simulink model "r2_b8a4x1kf"  (R2012b)
settings: Solver=VariableStepDiscrete  SolverMode=SingleTasking  StartTime=0.0  StopTime=1  RelTol=1e-3
undefined symbols (not defined in the file): fft_stages, n_bits_ants, n_bits_xengs
libraries: xbsIndex_r4 x22142, casper_library_misc x166, xbsReplacements_r4 x24, casper_library_delays x8, xps_library x5, casper_library_communications x4
(part 20 of 178)

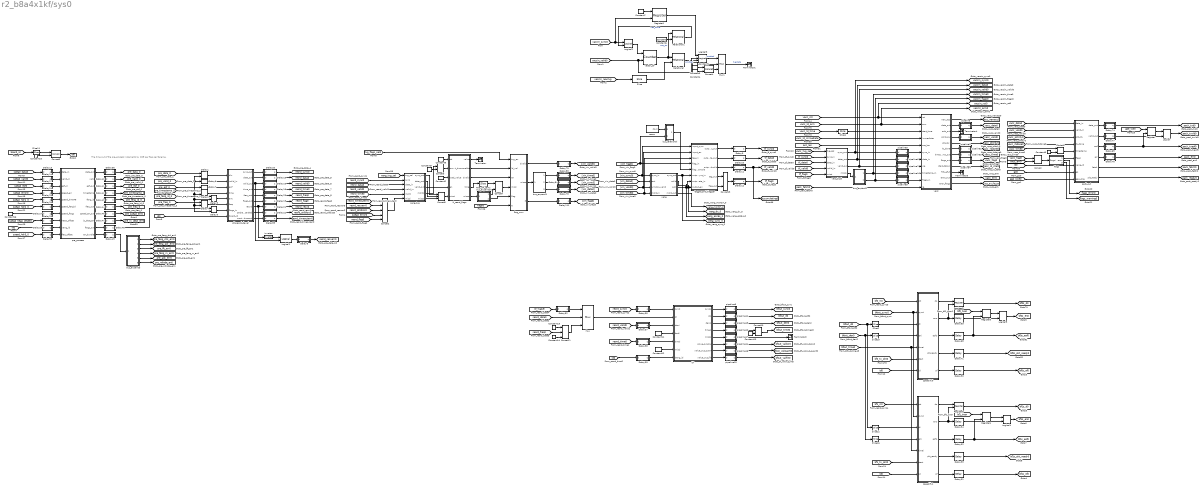
== system r2_b8a4x1kf/sys0 ==
  note: The time out of the pre_process increments
      | by ONE per freq per fengine.
  Concat{,1,3..4,6..7,10,13} (8 alike) : xbsIndex_r4/Concat  num_inputs=2  dbl_ovrd=off  block_type=concat
      Concat1 settings: block_version=10.1.3
      Concat4 settings: block_version=10.1.3
  Concat11 : xbsIndex_r4/Concat  num_inputs=3  dbl_ovrd=off  block_type=concat
  Concat2 : xbsIndex_r4/Concat  num_inputs=5  dbl_ovrd=off  block_type=concat
  Concat5 : xbsIndex_r4/Concat  num_inputs=3  dbl_ovrd=off  block_type=concat
  Constant1 : xbsIndex_r4/Constant  const=0  gui_display_data_type=Fixed-point  arith_type=Unsigned  n_bits=64  bin_pt=0  preci_type=Single  exp_width=8  frac_width=24  explicit_period=on  period=1  equ=P=C  opselect=C  inp2=PCIN>>17  opr=+  inp1=P  carry=CIN  dbl_ovrd=off  block_type=constant
  Constant10 : xbsIndex_r4/Constant  const=xeng_id  gui_display_data_type=Fixed-point  arith_type=Unsigned  n_bits=n_bits_xengs_per_fpga  bin_pt=0  preci_type=Single  exp_width=8  frac_width=24  explicit_period=on  period=1  equ=P=C  opselect=C  inp2=PCIN>>17  opr=+  inp1=P  carry=CIN  dbl_ovrd=off  block_type=constant
  Constant11 : xbsIndex_r4/Constant  const=0  gui_display_data_type=Fixed-point  arith_type=Boolean  n_bits=1  bin_pt=0  preci_type=Single  exp_width=8  frac_width=24  explicit_period=on  period=1  equ=P=C  opselect=C  inp2=PCIN>>17  opr=+  inp1=P  carry=CIN  dbl_ovrd=off  block_type=constant
      settings: block_version=11.3
  Constant12 : xbsIndex_r4/Constant  const=0  gui_display_data_type=Fixed-point  arith_type=Boolean  n_bits=1  bin_pt=0  preci_type=Single  exp_width=8  frac_width=24  explicit_period=on  period=1  equ=P=C  opselect=C  inp2=PCIN>>17  opr=+  inp1=P  carry=CIN  dbl_ovrd=off  block_type=constant
      settings: block_version=11.3
  Constant13 : xbsIndex_r4/Constant  const=0  gui_display_data_type=Fixed-point  arith_type=Unsigned  n_bits=n_bits_channels + 1 + x_acc_bits  bin_pt=0  preci_type=Single  exp_width=8  frac_width=24  explicit_period=on  period=1  equ=P=C  opselect=C  inp2=PCIN>>17  opr=+  inp1=P  carry=CIN  dbl_ovrd=off  block_type=constant
  Constant14 : xbsIndex_r4/Constant  const=0  gui_display_data_type=Fixed-point  arith_type=Unsigned  n_bits=16  bin_pt=0  preci_type=Single  exp_width=8  frac_width=24  explicit_period=on  period=1  equ=P=C  opselect=C  inp2=PCIN>>17  opr=+  inp1=P  carry=CIN  dbl_ovrd=off  block_type=constant
  Constant15 : xbsIndex_r4/Constant  const=0  gui_display_data_type=Fixed-point  arith_type=Unsigned  n_bits=16-n_bits_channels  bin_pt=0  preci_type=Single  exp_width=8  frac_width=24  explicit_period=on  period=1  equ=P=C  opselect=C  inp2=PCIN>>17  opr=+  inp1=P  carry=CIN  dbl_ovrd=off  block_type=constant
  Constant16 : xbsIndex_r4/Constant  const=0  gui_display_data_type=Fixed-point  arith_type=Unsigned  n_bits=48  bin_pt=0  preci_type=Single  exp_width=8  frac_width=24  explicit_period=on  period=1  equ=P=C  opselect=C  inp2=PCIN>>17  opr=+  inp1=P  carry=CIN  dbl_ovrd=off  block_type=constant
  Constant2 : xbsIndex_r4/Constant  const=0  gui_display_data_type=Boolean  arith_type=Boolean  n_bits=16  bin_pt=14  preci_type=Single  exp_width=8  frac_width=24  explicit_period=on  period=1  equ=P=C  opselect=C  inp2=PCIN>>17  opr=+  inp1=P  carry=CIN  dbl_ovrd=off  block_type=constant
  Constant3 : xbsIndex_r4/Constant  const=1  gui_display_data_type=Fixed-point  arith_type=Unsigned  n_bits=32  bin_pt=0  preci_type=Single  exp_width=8  frac_width=24  explicit_period=on  period=1  equ=P=C  opselect=C  inp2=PCIN>>17  opr=+  inp1=P  carry=CIN  dbl_ovrd=off  block_type=constant
  Constant4 : xbsIndex_r4/Constant  const=0  gui_display_data_type=Fixed-point  arith_type=Unsigned  n_bits=32  bin_pt=0  preci_type=Single  exp_width=8  frac_width=24  explicit_period=on  period=1  equ=P=C  opselect=C  inp2=PCIN>>17  opr=+  inp1=P  carry=CIN  dbl_ovrd=off  block_type=constant
  Constant5 : xbsIndex_r4/Constant  const=0  gui_display_data_type=Fixed-point  arith_type=Unsigned  n_bits=n_bits_channels + 1 + x_acc_bits  bin_pt=0  preci_type=Single  exp_width=8  frac_width=24  explicit_period=on  period=1  equ=P=C  opselect=C  inp2=PCIN>>17  opr=+  inp1=P  carry=CIN  dbl_ovrd=off  block_type=constant
  Constant6 : xbsIndex_r4/Constant  const=5120  gui_display_data_type=Fixed-point  arith_type=Unsigned  n_bits=13  bin_pt=0  preci_type=Single  exp_width=8  frac_width=24  explicit_period=on  period=1  equ=P=C  opselect=C  inp2=PCIN>>17  opr=+  inp1=P  carry=CIN  dbl_ovrd=off  block_type=constant
  Constant7 : xbsIndex_r4/Constant  const=1  gui_display_data_type=Boolean  arith_type=Boolean  n_bits=13  bin_pt=0  preci_type=Single  exp_width=8  frac_width=24  explicit_period=on  period=1  equ=P=C  opselect=C  inp2=PCIN>>17  opr=+  inp1=P  carry=CIN  dbl_ovrd=off  block_type=constant
  Constant8 : xbsIndex_r4/Constant  const=0  gui_display_data_type=Boolean  arith_type=Boolean  n_bits=16  bin_pt=14  preci_type=Single  exp_width=8  frac_width=24  explicit_period=on  period=1  equ=P=C  opselect=C  inp2=PCIN>>17  opr=+  inp1=P  carry=CIN  dbl_ovrd=off  block_type=constant
  Constant9 : xbsIndex_r4/Constant  const=0  gui_display_data_type=Fixed-point  arith_type=Unsigned  n_bits=n_bits_channels + 1 + x_acc_bits  bin_pt=0  preci_type=Single  exp_width=8  frac_width=24  explicit_period=on  period=1  equ=P=C  opselect=C  inp2=PCIN>>17  opr=+  inp1=P  carry=CIN  dbl_ovrd=off  block_type=constant
  Delay{1..5} (5 alike) : xbsIndex_r4/Delay  rst=off  infoeditControl=Selection of Reset will increase slice count due to use of real FFs and instead of SRLs  en=on  latency=1  dbl_ovrd=off  reg_retiming=on  block_type=delay
  Delay10 : Subsystem  AncestorBlock=casper_library_delays/pipeline  mask(pipeline){latency=2}
      mask help:
      | An explicitly laid-out delay line to avoid mapping to SRL16s
      | for use in pipelining to help achieve timing closure.
      mask init:
      | pipeline_init(gcb,'latency',latency);
      settings: AttributesFormatString=Latency = %<latency>
      mask Display:
      | port_label('input', 1, 'd');
      | port_label('output', 1, 'q');
      | disp(['Z^-', num2str(latency)]);
  Delay11 : Subsystem  AncestorBlock=casper_library_delays/pipeline  mask(pipeline){latency=2}
      mask help:
      | An explicitly laid-out delay line to avoid mapping to SRL16s
      | for use in pipelining to help achieve timing closure.
      mask init:
      | pipeline_init(gcb,'latency',latency);
      settings: AttributesFormatString=Latency = %<latency>
      mask Display:
      | port_label('input', 1, 'd');
      | port_label('output', 1, 'q');
      | disp(['Z^-', num2str(latency)]);
  Delay111 : Subsystem  AncestorBlock=casper_library_delays/pipeline  mask(pipeline){latency=2}
      mask help:
      | An explicitly laid-out delay line to avoid mapping to SRL16s
      | for use in pipelining to help achieve timing closure.
      mask init:
      | pipeline_init(gcb,'latency',latency);
      settings: AttributesFormatString=Latency = %<latency>
      mask Display:
      | port_label('input', 1, 'd');
      | port_label('output', 1, 'q');
      | disp(['Z^-', num2str(latency)]);
  Delay12 : Subsystem  AncestorBlock=casper_library_delays/pipeline  mask(pipeline){latency=2}
      mask help:
      | An explicitly laid-out delay line to avoid mapping to SRL16s
      | for use in pipelining to help achieve timing closure.
      mask init:
      | pipeline_init(gcb,'latency',latency);
      settings: AttributesFormatString=Latency = %<latency>
      mask Display:
      | port_label('input', 1, 'd');
      | port_label('output', 1, 'q');
      | disp(['Z^-', num2str(latency)]);
  Delay13 : Subsystem  AncestorBlock=casper_library_delays/pipeline  mask(pipeline){latency=2}
      mask help:
      | An explicitly laid-out delay line to avoid mapping to SRL16s
      | for use in pipelining to help achieve timing closure.
      mask init:
      | pipeline_init(gcb,'latency',latency);
      settings: AttributesFormatString=Latency = %<latency>
      mask Display:
      | port_label('input', 1, 'd');
      | port_label('output', 1, 'q');
      | disp(['Z^-', num2str(latency)]);
  Delay14 : Subsystem  AncestorBlock=casper_library_delays/pipeline  mask(pipeline){latency=2}
      mask help:
      | An explicitly laid-out delay line to avoid mapping to SRL16s
      | for use in pipelining to help achieve timing closure.
      mask init:
      | pipeline_init(gcb,'latency',latency);
      settings: AttributesFormatString=Latency = %<latency>
      mask Display:
      | port_label('input', 1, 'd');
      | port_label('output', 1, 'q');
      | disp(['Z^-', num2str(latency)]);
  Delay15 : Subsystem  AncestorBlock=casper_library_delays/pipeline  mask(pipeline){latency=2}
      mask help:
      | An explicitly laid-out delay line to avoid mapping to SRL16s
      | for use in pipelining to help achieve timing closure.
      mask init:
      | pipeline_init(gcb,'latency',latency);
      settings: AttributesFormatString=Latency = %<latency>
      mask Display:
      | port_label('input', 1, 'd');
      | port_label('output', 1, 'q');
      | disp(['Z^-', num2str(latency)]);
  Delay16 : Subsystem  AncestorBlock=casper_library_delays/pipeline  mask(pipeline){latency=2}
      mask help:
      | An explicitly laid-out delay line to avoid mapping to SRL16s
      | for use in pipelining to help achieve timing closure.
      mask init:
      | pipeline_init(gcb,'latency',latency);
      settings: AttributesFormatString=Latency = %<latency>
      mask Display:
      | port_label('input', 1, 'd');
      | port_label('output', 1, 'q');
      | disp(['Z^-', num2str(latency)]);
  Delay17 : Subsystem  AncestorBlock=casper_library_delays/pipeline  mask(pipeline){latency=2}
      mask help:
      | An explicitly laid-out delay line to avoid mapping to SRL16s
      | for use in pipelining to help achieve timing closure.
      mask init:
      | pipeline_init(gcb,'latency',latency);
      settings: AttributesFormatString=Latency = %<latency>
      mask Display:
      | port_label('input', 1, 'd');
      | port_label('output', 1, 'q');
      | disp(['Z^-', num2str(latency)]);
  Delay18 : Subsystem  AncestorBlock=casper_library_delays/pipeline  mask(pipeline){latency=2}
      mask help:
      | An explicitly laid-out delay line to avoid mapping to SRL16s
      | for use in pipelining to help achieve timing closure.
      mask init:
      | pipeline_init(gcb,'latency',latency);
      settings: AttributesFormatString=Latency = %<latency>
      mask Display:
      | port_label('input', 1, 'd');
      | port_label('output', 1, 'q');
      | disp(['Z^-', num2str(latency)]);
  Delay19 : Subsystem  AncestorBlock=casper_library_delays/pipeline  mask(pipeline){latency=2}
      mask help:
      | An explicitly laid-out delay line to avoid mapping to SRL16s
      | for use in pipelining to help achieve timing closure.
      mask init:
      | pipeline_init(gcb,'latency',latency);
      settings: AttributesFormatString=Latency = %<latency>
      mask Display:
      | port_label('input', 1, 'd');
      | port_label('output', 1, 'q');
      | disp(['Z^-', num2str(latency)]);
  Delay20 : Subsystem  AncestorBlock=casper_library_delays/pipeline  mask(pipeline){latency=2}
      mask help:
      | An explicitly laid-out delay line to avoid mapping to SRL16s
      | for use in pipelining to help achieve timing closure.
      mask init:
      | pipeline_init(gcb,'latency',latency);
      settings: AttributesFormatString=Latency = %<latency>
      mask Display:
      | port_label('input', 1, 'd');
      | port_label('output', 1, 'q');
      | disp(['Z^-', num2str(latency)]);
  Delay21 : Subsystem  AncestorBlock=casper_library_delays/pipeline  mask(pipeline){latency=2}
      mask help:
      | An explicitly laid-out delay line to avoid mapping to SRL16s
      | for use in pipelining to help achieve timing closure.
      mask init:
      | pipeline_init(gcb,'latency',latency);
      settings: AttributesFormatString=Latency = %<latency>
      mask Display:
      | port_label('input', 1, 'd');
      | port_label('output', 1, 'q');
      | disp(['Z^-', num2str(latency)]);
  Delay22 : Subsystem  AncestorBlock=casper_library_delays/pipeline  mask(pipeline){latency=2}
      mask help:
      | An explicitly laid-out delay line to avoid mapping to SRL16s
      | for use in pipelining to help achieve timing closure.
      mask init:
      | pipeline_init(gcb,'latency',latency);
      settings: AttributesFormatString=Latency = %<latency>
      mask Display:
      | port_label('input', 1, 'd');
      | port_label('output', 1, 'q');
      | disp(['Z^-', num2str(latency)]);
  Delay23 : Subsystem  AncestorBlock=casper_library_delays/pipeline  mask(pipeline){latency=2}
      mask help:
      | An explicitly laid-out delay line to avoid mapping to SRL16s
      | for use in pipelining to help achieve timing closure.
      mask init:
      | pipeline_init(gcb,'latency',latency);
      settings: AttributesFormatString=Latency = %<latency>
      mask Display:
      | port_label('input', 1, 'd');
      | port_label('output', 1, 'q');
      | disp(['Z^-', num2str(latency)]);
  Delay24 : Subsystem  AncestorBlock=casper_library_delays/pipeline  mask(pipeline){latency=2}
      mask help:
      | An explicitly laid-out delay line to avoid mapping to SRL16s
      | for use in pipelining to help achieve timing closure.
      mask init:
      | pipeline_init(gcb,'latency',latency);
      settings: AttributesFormatString=Latency = %<latency>
      mask Display:
      | port_label('input', 1, 'd');
      | port_label('output', 1, 'q');
      | disp(['Z^-', num2str(latency)]);
  Delay25 : Subsystem  AncestorBlock=casper_library_delays/pipeline  mask(pipeline){latency=2}
      mask help:
      | An explicitly laid-out delay line to avoid mapping to SRL16s
      | for use in pipelining to help achieve timing closure.
      mask init:
      | pipeline_init(gcb,'latency',latency);
      settings: AttributesFormatString=Latency = %<latency>
      mask Display:
      | port_label('input', 1, 'd');
      | port_label('output', 1, 'q');
      | disp(['Z^-', num2str(latency)]);
  Delay26 : Subsystem  AncestorBlock=casper_library_delays/pipeline  mask(pipeline){latency=2}
      mask help:
      | An explicitly laid-out delay line to avoid mapping to SRL16s
      | for use in pipelining to help achieve timing closure.
      mask init:
      | pipeline_init(gcb,'latency',latency);
      settings: AttributesFormatString=Latency = %<latency>
      mask Display:
      | port_label('input', 1, 'd');
      | port_label('output', 1, 'q');
      | disp(['Z^-', num2str(latency)]);
  Delay27 : Subsystem  AncestorBlock=casper_library_delays/pipeline  mask(pipeline){latency=2}
      mask help:
      | An explicitly laid-out delay line to avoid mapping to SRL16s
      | for use in pipelining to help achieve timing closure.
      mask init:
      | pipeline_init(gcb,'latency',latency);
      settings: AttributesFormatString=Latency = %<latency>
      mask Display:
      | port_label('input', 1, 'd');
      | port_label('output', 1, 'q');
      | disp(['Z^-', num2str(latency)]);
  Delay28 : Subsystem  AncestorBlock=casper_library_delays/pipeline  mask(pipeline){latency=2}
      mask help:
      | An explicitly laid-out delay line to avoid mapping to SRL16s
      | for use in pipelining to help achieve timing closure.
      mask init:
      | pipeline_init(gcb,'latency',latency);
      settings: AttributesFormatString=Latency = %<latency>
      mask Display:
      | port_label('input', 1, 'd');
      | port_label('output', 1, 'q');
      | disp(['Z^-', num2str(latency)]);
  Delay29 : Subsystem  AncestorBlock=casper_library_delays/pipeline  mask(pipeline){latency=2}
      mask help:
      | An explicitly laid-out delay line to avoid mapping to SRL16s
      | for use in pipelining to help achieve timing closure.
      mask init:
      | pipeline_init(gcb,'latency',latency);
      settings: AttributesFormatString=Latency = %<latency>
      mask Display:
      | port_label('input', 1, 'd');
      | port_label('output', 1, 'q');
      | disp(['Z^-', num2str(latency)]);
  Delay{6..7,30..34,68,71,93} (10 alike) : xbsIndex_r4/Delay  rst=off  infoeditControl=Selection of Reset will increase slice count due to use of real FFs and instead of SRLs  en=off  latency=1  dbl_ovrd=off  reg_retiming=on  block_type=delay
      Delay30 settings: block_version=11.4
      Delay31 settings: block_version=11.4
      Delay32 settings: block_version=11.4
      Delay33 settings: block_version=11.4
      Delay34 settings: block_version=11.4
      Delay68 settings: block_version=11.4
      Delay71 settings: block_version=11.4
      Delay93 settings: block_version=11.4
  Delay35 : Subsystem  AncestorBlock=casper_library_delays/pipeline  mask(pipeline){latency=1}
      mask help:
      | An explicitly laid-out delay line to avoid mapping to SRL16s
      | for use in pipelining to help achieve timing closure.
      mask init:
      | pipeline_init(gcb,'latency',latency);
      settings: AttributesFormatString=Latency = %<latency>
      mask Display:
      | port_label('input', 1, 'd');
      | port_label('output', 1, 'q');
      | disp(['Z^-', num2str(latency)]);
  Delay36 : Subsystem  AncestorBlock=casper_library_delays/pipeline  mask(pipeline){latency=2}
      mask help:
      | An explicitly laid-out delay line to avoid mapping to SRL16s
      | for use in pipelining to help achieve timing closure.
      mask init:
      | pipeline_init(gcb,'latency',latency);
      settings: AttributesFormatString=Latency = %<latency>
      mask Display:
      | port_label('input', 1, 'd');
      | port_label('output', 1, 'q');
      | disp(['Z^-', num2str(latency)]);
  Delay37 : Subsystem  AncestorBlock=casper_library_delays/pipeline  mask(pipeline){latency=1}
      mask help:
      | An explicitly laid-out delay line to avoid mapping to SRL16s
      | for use in pipelining to help achieve timing closure.
      mask init:
      | pipeline_init(gcb,'latency',latency);
      settings: AttributesFormatString=Latency = %<latency>
      mask Display:
      | port_label('input', 1, 'd');
      | port_label('output', 1, 'q');
      | disp(['Z^-', num2str(latency)]);
  Delay38 : Subsystem  AncestorBlock=casper_library_delays/pipeline  mask(pipeline){latency=1}
      mask help:
      | An explicitly laid-out delay line to avoid mapping to SRL16s
      | for use in pipelining to help achieve timing closure.
      mask init:
      | pipeline_init(gcb,'latency',latency);
      settings: AttributesFormatString=Latency = %<latency>
      mask Display:
      | port_label('input', 1, 'd');
      | port_label('output', 1, 'q');
      | disp(['Z^-', num2str(latency)]);
  Delay39 : Subsystem  AncestorBlock=casper_library_delays/pipeline  mask(pipeline){latency=1}
      mask help:
      | An explicitly laid-out delay line to avoid mapping to SRL16s
      | for use in pipelining to help achieve timing closure.
      mask init:
      | pipeline_init(gcb,'latency',latency);
      settings: AttributesFormatString=Latency = %<latency>
      mask Display:
      | port_label('input', 1, 'd');
      | port_label('output', 1, 'q');
      | disp(['Z^-', num2str(latency)]);
  Delay40 : Subsystem  AncestorBlock=casper_library_delays/pipeline  mask(pipeline){latency=2}
      mask help:
      | An explicitly laid-out delay line to avoid mapping to SRL16s
      | for use in pipelining to help achieve timing closure.
      mask init:
      | pipeline_init(gcb,'latency',latency);
      settings: AttributesFormatString=Latency = %<latency>
      mask Display:
      | port_label('input', 1, 'd');
      | port_label('output', 1, 'q');
      | disp(['Z^-', num2str(latency)]);
  Delay41 : Subsystem  AncestorBlock=casper_library_delays/pipeline  mask(pipeline){latency=2}
      mask help:
      | An explicitly laid-out delay line to avoid mapping to SRL16s
      | for use in pipelining to help achieve timing closure.
      mask init:
      | pipeline_init(gcb,'latency',latency);
      settings: AttributesFormatString=Latency = %<latency>
      mask Display:
      | port_label('input', 1, 'd');
      | port_label('output', 1, 'q');
      | disp(['Z^-', num2str(latency)]);
  Delay42 : Subsystem  AncestorBlock=casper_library_delays/pipeline  mask(pipeline){latency=2}
      mask help:
      | An explicitly laid-out delay line to avoid mapping to SRL16s
      | for use in pipelining to help achieve timing closure.
      mask init:
      | pipeline_init(gcb,'latency',latency);
      settings: AttributesFormatString=Latency = %<latency>
      mask Display:
      | port_label('input', 1, 'd');
      | port_label('output', 1, 'q');
      | disp(['Z^-', num2str(latency)]);
  Delay43 : Subsystem  AncestorBlock=casper_library_delays/pipeline  mask(pipeline){latency=2}
      mask help:
      | An explicitly laid-out delay line to avoid mapping to SRL16s
      | for use in pipelining to help achieve timing closure.
      mask init:
      | pipeline_init(gcb,'latency',latency);
      settings: AttributesFormatString=Latency = %<latency>
      mask Display:
      | port_label('input', 1, 'd');
      | port_label('output', 1, 'q');
      | disp(['Z^-', num2str(latency)]);
  Delay44 : Subsystem  AncestorBlock=casper_library_delays/pipeline  mask(pipeline){latency=2}
      mask help:
      | An explicitly laid-out delay line to avoid mapping to SRL16s
      | for use in pipelining to help achieve timing closure.
      mask init:
      | pipeline_init(gcb,'latency',latency);
      settings: AttributesFormatString=Latency = %<latency>
      mask Display:
      | port_label('input', 1, 'd');
      | port_label('output', 1, 'q');
      | disp(['Z^-', num2str(latency)]);
  Delay46 : Subsystem  AncestorBlock=casper_library_delays/pipeline  mask(pipeline){latency=2}
      mask help:
      | An explicitly laid-out delay line to avoid mapping to SRL16s
      | for use in pipelining to help achieve timing closure.
      mask init:
      | pipeline_init(gcb,'latency',latency);
      settings: AttributesFormatString=Latency = %<latency>
      mask Display:
      | port_label('input', 1, 'd');
      | port_label('output', 1, 'q');
      | disp(['Z^-', num2str(latency)]);
  Delay47 : Subsystem  AncestorBlock=casper_library_delays/pipeline  mask(pipeline){latency=2}
      mask help:
      | An explicitly laid-out delay line to avoid mapping to SRL16s
      | for use in pipelining to help achieve timing closure.
      mask init:
      | pipeline_init(gcb,'latency',latency);
      settings: AttributesFormatString=Latency = %<latency>
      mask Display:
      | port_label('input', 1, 'd');
      | port_label('output', 1, 'q');
      | disp(['Z^-', num2str(latency)]);
  Delay48 : Subsystem  AncestorBlock=casper_library_delays/pipeline  mask(pipeline){latency=2}
      mask help:
      | An explicitly laid-out delay line to avoid mapping to SRL16s
      | for use in pipelining to help achieve timing closure.
      mask init:
      | pipeline_init(gcb,'latency',latency);
      settings: AttributesFormatString=Latency = %<latency>
      mask Display:
      | port_label('input', 1, 'd');
      | port_label('output', 1, 'q');
      | disp(['Z^-', num2str(latency)]);
  Delay49 : Subsystem  AncestorBlock=casper_library_delays/pipeline  mask(pipeline){latency=2}
      mask help:
      | An explicitly laid-out delay line to avoid mapping to SRL16s
      | for use in pipelining to help achieve timing closure.
      mask init:
      | pipeline_init(gcb,'latency',latency);
      settings: AttributesFormatString=Latency = %<latency>
      mask Display:
      | port_label('input', 1, 'd');
      | port_label('output', 1, 'q');
      | disp(['Z^-', num2str(latency)]);
  Delay50 : Subsystem  AncestorBlock=casper_library_delays/pipeline  mask(pipeline){latency=2}
      mask help:
      | An explicitly laid-out delay line to avoid mapping to SRL16s
      | for use in pipelining to help achieve timing closure.
      mask init:
      | pipeline_init(gcb,'latency',latency);
      settings: AttributesFormatString=Latency = %<latency>
      mask Display:
      | port_label('input', 1, 'd');
      | port_label('output', 1, 'q');
      | disp(['Z^-', num2str(latency)]);
  Delay52 : Subsystem  AncestorBlock=casper_library_delays/pipeline  mask(pipeline){latency=1}
      mask help:
      | An explicitly laid-out delay line to avoid mapping to SRL16s
      | for use in pipelining to help achieve timing closure.
      mask init:
      | pipeline_init(gcb,'latency',latency);
      settings: AttributesFormatString=Latency = %<latency>
      mask Display:
      | port_label('input', 1, 'd');
      | port_label('output', 1, 'q');
      | disp(['Z^-', num2str(latency)]);
  Delay69 : Subsystem  AncestorBlock=casper_library_delays/pipeline  mask(pipeline){latency=2}
      mask help:
      | An explicitly laid-out delay line to avoid mapping to SRL16s
      | for use in pipelining to help achieve timing closure.
      mask init:
      | pipeline_init(gcb,'latency',latency);
      settings: AttributesFormatString=Latency = %<latency>
      mask Display:
      | port_label('input', 1, 'd');
      | port_label('output', 1, 'q');
      | disp(['Z^-', num2str(latency)]);
  Delay74 : Subsystem  AncestorBlock=casper_library_delays/pipeline  mask(pipeline){latency=2}
      mask help:
      | An explicitly laid-out delay line to avoid mapping to SRL16s
      | for use in pipelining to help achieve timing closure.
      mask init:
      | pipeline_init(gcb,'latency',latency);
      settings: AttributesFormatString=Latency = %<latency>
      mask Display:
      | port_label('input', 1, 'd');
      | port_label('output', 1, 'q');
      | disp(['Z^-', num2str(latency)]);
  Delay76 : Subsystem  AncestorBlock=casper_library_delays/pipeline  mask(pipeline){latency=2}
      mask help:
      | An explicitly laid-out delay line to avoid mapping to SRL16s
      | for use in pipelining to help achieve timing closure.
      mask init:
      | pipeline_init(gcb,'latency',latency);
      settings: AttributesFormatString=Latency = %<latency>
      mask Display:
      | port_label('input', 1, 'd');
      | port_label('output', 1, 'q');
      | disp(['Z^-', num2str(latency)]);
  Delay77 : Subsystem  AncestorBlock=casper_library_delays/pipeline  mask(pipeline){latency=2}
      mask help:
      | An explicitly laid-out delay line to avoid mapping to SRL16s
      | for use in pipelining to help achieve timing closure.
      mask init:
      | pipeline_init(gcb,'latency',latency);
      settings: AttributesFormatString=Latency = %<latency>
      mask Display:
      | port_label('input', 1, 'd');
      | port_label('output', 1, 'q');
      | disp(['Z^-', num2str(latency)]);
  Delay78 : Subsystem  AncestorBlock=casper_library_delays/pipeline  mask(pipeline){latency=2}
      mask help:
      | An explicitly laid-out delay line to avoid mapping to SRL16s
      | for use in pipelining to help achieve timing closure.
      mask init:
      | pipeline_init(gcb,'latency',latency);
      settings: AttributesFormatString=Latency = %<latency>
      mask Display:
      | port_label('input', 1, 'd');
      | port_label('output', 1, 'q');
      | disp(['Z^-', num2str(latency)]);
  Delay79 : Subsystem  AncestorBlock=casper_library_delays/pipeline  mask(pipeline){latency=2}
      mask help:
      | An explicitly laid-out delay line to avoid mapping to SRL16s
      | for use in pipelining to help achieve timing closure.
      mask init:
      | pipeline_init(gcb,'latency',latency);
      settings: AttributesFormatString=Latency = %<latency>
      mask Display:
      | port_label('input', 1, 'd');
      | port_label('output', 1, 'q');
      | disp(['Z^-', num2str(latency)]);
  Delay8 : Subsystem  AncestorBlock=casper_library_delays/pipeline  mask(pipeline){latency=1}
      mask help:
      | An explicitly laid-out delay line to avoid mapping to SRL16s
      | for use in pipelining to help achieve timing closure.
      mask init:
      | pipeline_init(gcb,'latency',latency);
      settings: AttributesFormatString=Latency = %<latency>
      mask Display:
      | port_label('input', 1, 'd');
      | port_label('output', 1, 'q');
      | disp(['Z^-', num2str(latency)]);
  Delay83 : Subsystem  AncestorBlock=casper_library_delays/pipeline  mask(pipeline){latency=2}
      mask help:
      | An explicitly laid-out delay line to avoid mapping to SRL16s
      | for use in pipelining to help achieve timing closure.
      mask init:
      | pipeline_init(gcb,'latency',latency);
      settings: AttributesFormatString=Latency = %<latency>
      mask Display:
      | port_label('input', 1, 'd');
      | port_label('output', 1, 'q');
      | disp(['Z^-', num2str(latency)]);
  Delay84 : Subsystem  AncestorBlock=casper_library_delays/pipeline  mask(pipeline){latency=2}
      mask help:
      | An explicitly laid-out delay line to avoid mapping to SRL16s
      | for use in pipelining to help achieve timing closure.
      mask init:
      | pipeline_init(gcb,'latency',latency);
      settings: AttributesFormatString=Latency = %<latency>
      mask Display:
      | port_label('input', 1, 'd');
      | port_label('output', 1, 'q');
      | disp(['Z^-', num2str(latency)]);
  Delay89 : Subsystem  AncestorBlock=casper_library_delays/pipeline  mask(pipeline){latency=2}
      mask help:
      | An explicitly laid-out delay line to avoid mapping to SRL16s
      | for use in pipelining to help achieve timing closure.
      mask init:
      | pipeline_init(gcb,'latency',latency);
      settings: AttributesFormatString=Latency = %<latency>
      mask Display:
      | port_label('input', 1, 'd');
      | port_label('output', 1, 'q');
      | disp(['Z^-', num2str(latency)]);
  Delay9 : Subsystem  AncestorBlock=casper_library_delays/pipeline  mask(pipeline){latency=2}
      mask help:
      | An explicitly laid-out delay line to avoid mapping to SRL16s
      | for use in pipelining to help achieve timing closure.
      mask init:
      | pipeline_init(gcb,'latency',latency);
      settings: AttributesFormatString=Latency = %<latency>
      mask Display:
      | port_label('input', 1, 'd');
      | port_label('output', 1, 'q');
      | disp(['Z^-', num2str(latency)]);
  Inverter : xbsIndex_r4/Inverter  en=off  latency=0  dbl_ovrd=off  block_type=inv
  Logical : xbsIndex_r4/Logical  logical_function=AND  inputs=2  en=off  latency=0  precision=Full  arith_type=Unsigned  n_bits=16  bin_pt=0  align_bp=on  dbl_ovrd=off  block_type=logical
  Logical1 : xbsIndex_r4/Logical  logical_function=AND  inputs=2  en=off  latency=1  precision=Full  arith_type=Unsigned  n_bits=16  bin_pt=0  align_bp=on  dbl_ovrd=off  block_type=logical
  Logical2 : xbsIndex_r4/Logical  logical_function=OR  inputs=2  en=off  latency=0  precision=Full  arith_type=Unsigned  n_bits=16  bin_pt=0  align_bp=on  dbl_ovrd=off  block_type=logical
  Logical3 : xbsIndex_r4/Logical  logical_function=AND  inputs=3  en=off  latency=0  precision=Full  arith_type=Unsigned  n_bits=16  bin_pt=0  align_bp=on  dbl_ovrd=off  block_type=logical
  Logical4 : xbsIndex_r4/Logical  logical_function=AND  inputs=2  en=off  latency=0  precision=Full  arith_type=Unsigned  n_bits=16  bin_pt=0  align_bp=on  dbl_ovrd=off  block_type=logical
  Logical5 : xbsIndex_r4/Logical  logical_function=AND  inputs=2  en=off  latency=0  precision=Full  arith_type=Unsigned  n_bits=16  bin_pt=0  align_bp=on  dbl_ovrd=off  block_type=logical
  Mux : xbsIndex_r4/Mux  inputs=2  en=off  latency=1  precision=Full  arith_type=Unsigned  n_bits=16  bin_pt=14  quantization=Truncate  overflow=Wrap  dbl_ovrd=off  block_type=mux
  Mux1 : xbsIndex_r4/Mux  inputs=2  en=off  latency=0  precision=Full  arith_type=Unsigned  n_bits=16  bin_pt=14  quantization=Truncate  overflow=Wrap  dbl_ovrd=off  block_type=mux
  Register{,1..5} (6 alike) : xbsIndex_r4/Register  init=0  rst=off  en=on  dbl_ovrd=off  block_type=register
      Register2 settings: block_version=11.4
      Register3 settings: block_version=11.4
  Relational : xbsIndex_r4/Relational  mode=a=b  en=off  latency=0  dbl_ovrd=off  block_type=relational
  Relational1 : xbsIndex_r4/Relational  mode=a=b  en=off  latency=0  dbl_ovrd=off  block_type=relational
  Slice : xbsIndex_r4/Slice  nbits=13  boolean_output=off  mode=Lower Bit Location + Width  bit1=0  base1=MSB of Input  bit0=0  base0=LSB of Input  dbl_ovrd=off  block_type=slice
  Slice1 : xbsIndex_r4/Slice  nbits=timestamp_bits  boolean_output=off  mode=Upper Bit Location + Width  bit1=0  base1=MSB of Input  bit0=timestamp_bits  base0=LSB of Input  dbl_ovrd=off  block_type=slice
  Slice11 : xbsIndex_r4/Slice  nbits=n_bits_xengs - n_bits_xengs_per_fpga  boolean_output=off  mode=Lower Bit Location + Width  bit1=0  base1=MSB of Input  bit0=0  base0=LSB of Input  dbl_ovrd=off  block_type=slice
      settings: block_version=10.1.3
  Slice12 : xbsIndex_r4/Slice  nbits=16  boolean_output=off  mode=Lower Bit Location + Width  bit1=0  base1=MSB of Input  bit0=0  base0=LSB of Input  dbl_ovrd=off  block_type=slice
  Slice15 : xbsIndex_r4/Slice  nbits=1  boolean_output=on  mode=Upper Bit Location + Width  bit1=0  base1=MSB of Input  bit0=0  base0=LSB of Input  dbl_ovrd=off  block_type=slice
  Slice16 : xbsIndex_r4/Slice  nbits=1  boolean_output=on  mode=Lower Bit Location + Width  bit1=0  base1=LSB of Input  bit0=0  base0=LSB of Input  dbl_ovrd=off  block_type=slice
  Slice2 : xbsIndex_r4/Slice  nbits=16  boolean_output=off  mode=Upper Bit Location + Width  bit1=0  base1=MSB of Input  bit0=0  base0=LSB of Input  dbl_ovrd=off  block_type=slice
  Terminator{,1..2,4..5} (5 alike) : Terminator
  bf : Subsystem  mask{beng_bits=n_bits_xengs, ant_bits=n_bits_ants, polarisation_bits=1, freq_bits=n_bits_channels, stack_bits=x_acc_bits, n_bits_in=8, bin_pt_in=7, bfpga_bits=2, timestamp_bits=timestamp_bits, n_bits_norm=16, bin_pt_norm=9, n_bits_combine=8+16+1+n_bits_ants, n_bits_requant=16, bin_pt_requant=8, bram_latency=5, add_latency=3, mult_latency=5, beam_bits=0, n_bits_out=8, bin_pt_out=7, conv_latency=3, output_enabled=off}
      mask prompts: beng_bits "b-engines (2^?)"; ant_bits "antennas (2^?)"; polarisation_bits "polarisations (2^?)"; freq_bits "frequencies (2^?)"; stack_bits "stacking factor (2^?)"; n_bits_in "data bits in"; bin_pt_in "binary point in"; bfpga_bits "b-engines on FPGA"; timestamp_bits "timestamp size (bits)"; n_bits_norm "calibration factor data bits"; bin_pt_norm "calibration factor binary point"; n_bits_combine "antenna combination output bit width"; n_bits_requant "requantization factor bit width"; bin_pt_requant "requantization factor binary point"; bram_latency "bram latency"; add_latency "add latency"; beam_bits "beams (2^?)"; n_bits_out "data bits out"; bin_pt_out "binary point out"; conv_latency "convert latency"; output_enabled "output enabled by default?"
      mask help:
      | Frequency domain beamformer
      |
      | b-engines: number of b-engines in system (same as x-engines)
      | stacking factor: the number of consecutive time samples in a data block
      | calibration factor: the complex factor multiplied with the incoming data.
      | The complex value is unique to each beam, input and frequency.
      | Requantization factor: real factor multiplied with the output data before
      | quantization. The value is unique to each beam and frequency.
      | beams: the number of beams per polarisation
      | ouput enabled by default: can be useful for simulation
      mask init:
      | set_param([gcb,'/fbf'], ...
      |     'output_enabled', output_enabled);
      mask Help:
      | Accepts the same channelised data as the CASPER FX correlator x-engine core.
      | Polarisations appear in order in different beams. (for polarisation (0,1), 0 in [0,2...], 1 in [1,3...]).
      | TODO: beam steering.
      | TODO: Stokes output.
      | TODO: accumulation.
  bus_expand1 : Subsystem  AncestorBlock=casper_library_flow_control/bus_expand  mask(bus_expand){mode=divisions of arbitrary size, outputNum=1, outputWidth=[timestamp_bits 1 (8*2*2)], outputBinaryPt=[0 0 0], outputArithmeticType=[0 2 0], outputToWorkspace=off, variablePrefix=out, outputToModelAsWell=on}
      mask prompts: outputNum "Number of outputs:"; outputWidth "Output width [msb ... lsb]:"; outputBinaryPt "Output binary point position [msb ... lsb]:"; outputArithmeticType "Output arithmetic type (ufix=0, fix=1, bool=2) [msb ... lsb]:"; outputToWorkspace "Output to workspace?"; variablePrefix "Variable name prefix:"; outputToModelAsWell "Output to model as well?"
      mask help:
      | Expands a 'bus' made using a bus_create or Xilinx
      | concat block.
      | The input will be divided into the specified number
      | of outputs with the specified arithmetic types.
      | Divisions are made from most significant bit.
      mask init:
      | bus_expand_init(gcb,...
      |     'mode', mode, ...
      |     'outputNum', outputNum, ...
      |     'outputWidth', outputWidth, ...
      |     'outputBinaryPt', outputBinaryPt, ...
      |     'outputArithmeticType', outputArithmeticType, ...
      |     'outputToWorkspace', outputToWorkspace, ...
      |     'variablePrefix', variablePrefix, ...
      |     'outputToModelAsWell', outputToModelAsWell);
      settings: AttributesFormatString=3 outputs
      mask TypeOptions mode: divisions of equal size | divisions of arbitrary size
      mask Callback mode: bus_expand_callback();
      mask Callback outputWidth: bus_expand_callback();
      mask Callback outputToWorkspace: bus_expand_callback();
  bus_expand2 : Subsystem  AncestorBlock=casper_library_flow_control/bus_expand  mask(bus_expand){mode=divisions of arbitrary size, outputNum=1, outputWidth=[timestamp_bits, 19], outputBinaryPt=[0 0], outputArithmeticType=[0 0], show_format=on, outputToWorkspace=off, variablePrefix=out, outputToModelAsWell=on}
      mask prompts: outputNum "Number of outputs:"; outputWidth "Output width [msb ... lsb]:"; outputBinaryPt "Output binary point position [msb ... lsb]:"; outputArithmeticType "Output arithmetic type (ufix=0, fix=1, bool=2) [msb ... lsb]:"; show_format "Print format string?"; outputToWorkspace "Output to workspace?"; variablePrefix "Variable name prefix:"; outputToModelAsWell "Output to model as well?"
      mask help:
      | Expands a 'bus' made using a bus_create or Xilinx
      | concat block.
      | The input will be divided into the specified number
      | of outputs with the specified arithmetic types.
      | Divisions are made from most significant bit.
      mask init: same as r2_b8a4x1kf/bus_expand
      settings: AttributesFormatString=2 outputs: uf24.0,uf19.0,
      mask TypeOptions mode: divisions of equal size | divisions of arbitrary size
      mask Callback mode: bus_expand_callback();
      mask Callback outputWidth: bus_expand_callback();
      mask Callback outputToWorkspace: bus_expand_callback();
  bus_expand20 : Subsystem  AncestorBlock=casper_library_flow_control/bus_expand  mask(bus_expand){mode=divisions of arbitrary size, outputNum=1, outputWidth=[(8*2*2+1) 19], outputBinaryPt=[0 0], outputArithmeticType=[0 0], outputToWorkspace=off, variablePrefix=out, outputToModelAsWell=on}
      mask prompts: outputNum "Number of outputs:"; outputWidth "Output width [msb ... lsb]:"; outputBinaryPt "Output binary point position [msb ... lsb]:"; outputArithmeticType "Output arithmetic type (ufix=0, fix=1, bool=2) [msb ... lsb]:"; outputToWorkspace "Output to workspace?"; variablePrefix "Variable name prefix:"; outputToModelAsWell "Output to model as well?"
      mask help:
      | Expands a 'bus' made using a bus_create or Xilinx
      | concat block.
      | The input will be divided into the specified number
      | of outputs with the specified arithmetic types.
      | Divisions are made from most significant bit.
      mask init: same as r2_b8a4x1kf/sys0/bus_expand1
      settings: AttributesFormatString=2 outputs
      mask TypeOptions mode: divisions of equal size | divisions of arbitrary size
      mask Callback mode: bus_expand_callback();
      mask Callback outputWidth: bus_expand_callback();
      mask Callback outputToWorkspace: bus_expand_callback();
  bus_expand3 : Subsystem  AncestorBlock=casper_library_flow_control/bus_expand  mask(bus_expand){mode=divisions of equal size, outputNum=6, outputWidth=1, outputBinaryPt=0, outputArithmeticType=2, show_format=on, outputToWorkspace=off, variablePrefix=out, outputToModelAsWell=on}
      mask prompts: outputNum "Number of outputs:"; outputWidth "Output width:"; outputBinaryPt "Output binary point position:"; outputArithmeticType "Output arithmetic type (ufix=0, fix=1, bool=2):"; show_format "Print format string?"; outputToWorkspace "Output to workspace?"; variablePrefix "Variable name prefix:"; outputToModelAsWell "Output to model as well?"
      mask help:
      | Expands a 'bus' made using a bus_create or Xilinx
      | concat block.
      | The input will be divided into the specified number
      | of outputs with the specified arithmetic types.
      | Divisions are made from most significant bit.
      mask init: same as r2_b8a4x1kf/bus_expand
      settings: AttributesFormatString=6 outputs: b,b,b,b,b,b,
      mask TypeOptions mode: divisions of equal size | divisions of arbitrary size
      mask Callback mode: bus_expand_callback();
      mask Callback outputWidth: bus_expand_callback();
      mask Callback outputToWorkspace: bus_expand_callback();
  bus_relational : Subsystem  AncestorBlock=casper_library_bus/bus_relational  mask(bus_relational){n_bits_a=ones(1,19), bin_pt_a=0, type_a=0, n_bits_b=ones(1,19), bin_pt_b=0, type_b=0, en=off, misc=off, mode=a!=b, latency=0}
      mask prompts: n_bits_a "a input bit widths"; bin_pt_a "a input binary points"; type_a "a input type (Unsigned=0, Signed=1)"; n_bits_b "b input bit widths"; bin_pt_b "b input binary points"; type_b "b input type (Unsigned=0, Signed=1)"; en "en port"; misc "misc support"; mode "comparison:"
      mask help: Find the relational product of two busses
      mask init:
      | bus_relational_init(gcb, ...
      |     'n_bits_a', n_bits_a, ...
      |     'bin_pt_a', bin_pt_a, ...
      |     'type_a', type_a, ...
      |     'n_bits_b', n_bits_b, ...
      |     'bin_pt_b', bin_pt_b, ...
      |     'type_b', type_b, ...
      |     'en', en, ...
      |     'misc', misc, ...
      |     'mode', mode, ...
      |     'latency', latency);
      mask TypeOptions mode: a=b | a!=b | a<b | a>b | a<=b | a>=b
  flag_mux : Subsystem  mask{n_bits=19}
      mask prompts: n_bits "flag bitwidth"
  flags : Subsystem
  pack_out : Subsystem  mask(pkt_pack_mask){vector_len=(2^n_bits_ants*(2^n_bits_ants+1))/2*8*2^(n_bits_channels-n_bits_xengs-1), n_bits_chans=n_bits_channels-n_bits_xengs, n_bits_word_size=3, heap_len=(2^n_bits_ants*(2^n_bits_ants+1))/2*8*(2^(n_bits_channels-n_bits_xengs))*4, fifo_latency=3, spead_msw=64, spead_lsw=48, spead_item=6144, pkt_bits=9, n_bits_max_gap=20, n_bits_timestamp_padding=((n_bits_channels + 1 + x_acc_bits)-3)+3}
      mask prompts: vector_len "vector length (words)"; n_bits_chans "frequency channels (2^?)"; n_bits_word_size "word size (2^? bytes)"; heap_len "System heap size (bytes)"; fifo_latency "Fifo Latency"; spead_msw "SPEAD flavour (MSw)"; spead_lsw "SPEAD flavour (LSw)"; spead_item "SPEAD item number"; pkt_bits "desired payload length (2^?) 64-bit words"; n_bits_max_gap "max gap between packets (2^? clock cycles)"; n_bits_timestamp_padding "Timestamp padding"
      mask help:
      | This block generates packets from a datastream.
      |
      | Packets are created with a fixed header followed by a user-specified number of 64-bit options.
      |
      | Requires a 64-bit data stream.
      |
      | System head size: number of baselines * number of stokes values * number of words per stokes value * number of frequencies * number of bytes per word
      |
      | See the documentation for further details.
      mask init:
      | vector_bits = ceil(log2(vector_len));
      | pkt_len=2^(pkt_bits);
  pipeline : Subsystem  AncestorBlock=casper_library_delays/pipeline  mask(pipeline){latency=2}
      mask help:
      | An explicitly laid-out delay line to avoid mapping to SRL16s
      | for use in pipelining to help achieve timing closure.
      mask init:
      | pipeline_init(gcb,'latency',latency);
      settings: AttributesFormatString=Latency = %<latency>
      mask Display:
      | port_label('input', 1, 'd');
      | port_label('output', 1, 'q');
      | disp(['Z^-', num2str(latency)]);
  pipeline1 : Subsystem  AncestorBlock=casper_library_delays/pipeline  mask(pipeline){latency=2}
      mask help:
      | An explicitly laid-out delay line to avoid mapping to SRL16s
      | for use in pipelining to help achieve timing closure.
      mask init:
      | pipeline_init(gcb,'latency',latency);
      settings: AttributesFormatString=Latency = %<latency>
      mask Display:
      | port_label('input', 1, 'd');
      | port_label('output', 1, 'q');
      | disp(['Z^-', num2str(latency)]);
  pipeline10 : Subsystem  AncestorBlock=casper_library_delays/pipeline  mask(pipeline){latency=2}
      mask help:
      | An explicitly laid-out delay line to avoid mapping to SRL16s
      | for use in pipelining to help achieve timing closure.
      mask init:
      | pipeline_init(gcb,'latency',latency);
      settings: AttributesFormatString=Latency = %<latency>
      mask Display:
      | port_label('input', 1, 'd');
      | port_label('output', 1, 'q');
      | disp(['Z^-', num2str(latency)]);
  pipeline11 : Subsystem  AncestorBlock=casper_library_delays/pipeline  mask(pipeline){latency=4}
      mask help:
      | An explicitly laid-out delay line to avoid mapping to SRL16s
      | for use in pipelining to help achieve timing closure.
      mask init:
      | pipeline_init(gcb,'latency',latency);
      settings: AttributesFormatString=Latency = %<latency>
      mask Display:
      | port_label('input', 1, 'd');
      | port_label('output', 1, 'q');
      | disp(['Z^-', num2str(latency)]);
  pipeline12 : Subsystem  AncestorBlock=casper_library_delays/pipeline  mask(pipeline){latency=4}
      mask help:
      | An explicitly laid-out delay line to avoid mapping to SRL16s
      | for use in pipelining to help achieve timing closure.
      mask init:
      | pipeline_init(gcb,'latency',latency);
      settings: AttributesFormatString=Latency = %<latency>
      mask Display:
      | port_label('input', 1, 'd');
      | port_label('output', 1, 'q');
      | disp(['Z^-', num2str(latency)]);
  pipeline13 : Subsystem  AncestorBlock=casper_library_delays/pipeline  mask(pipeline){latency=4}
      mask help:
      | An explicitly laid-out delay line to avoid mapping to SRL16s
      | for use in pipelining to help achieve timing closure.
      mask init:
      | pipeline_init(gcb,'latency',latency);
      settings: AttributesFormatString=Latency = %<latency>
      mask Display:
      | port_label('input', 1, 'd');
      | port_label('output', 1, 'q');
      | disp(['Z^-', num2str(latency)]);
  pipeline14 : Subsystem  AncestorBlock=casper_library_delays/pipeline  mask(pipeline){latency=4}
      mask help:
      | An explicitly laid-out delay line to avoid mapping to SRL16s
      | for use in pipelining to help achieve timing closure.
      mask init:
      | pipeline_init(gcb,'latency',latency);
      settings: AttributesFormatString=Latency = %<latency>
      mask Display:
      | port_label('input', 1, 'd');
      | port_label('output', 1, 'q');
      | disp(['Z^-', num2str(latency)]);
  pipeline15 : Subsystem  AncestorBlock=casper_library_delays/pipeline  mask(pipeline){latency=4}
      mask help:
      | An explicitly laid-out delay line to avoid mapping to SRL16s
      | for use in pipelining to help achieve timing closure.
      mask init:
      | pipeline_init(gcb,'latency',latency);
      settings: AttributesFormatString=Latency = %<latency>
      mask Display:
      | port_label('input', 1, 'd');
      | port_label('output', 1, 'q');
      | disp(['Z^-', num2str(latency)]);
  pipeline16 : Subsystem  AncestorBlock=casper_library_delays/pipeline  mask(pipeline){latency=4}
      mask help:
      | An explicitly laid-out delay line to avoid mapping to SRL16s
      | for use in pipelining to help achieve timing closure.
      mask init:
      | pipeline_init(gcb,'latency',latency);
      settings: AttributesFormatString=Latency = %<latency>
      mask Display:
      | port_label('input', 1, 'd');
      | port_label('output', 1, 'q');
      | disp(['Z^-', num2str(latency)]);
  pipeline17 : Subsystem  AncestorBlock=casper_library_delays/pipeline  mask(pipeline){latency=4}
      mask help:
      | An explicitly laid-out delay line to avoid mapping to SRL16s
      | for use in pipelining to help achieve timing closure.
      mask init:
      | pipeline_init(gcb,'latency',latency);
      settings: AttributesFormatString=Latency = %<latency>
      mask Display:
      | port_label('input', 1, 'd');
      | port_label('output', 1, 'q');
      | disp(['Z^-', num2str(latency)]);
  pipeline2 : Subsystem  AncestorBlock=casper_library_delays/pipeline  mask(pipeline){latency=2}
      mask help:
      | An explicitly laid-out delay line to avoid mapping to SRL16s
      | for use in pipelining to help achieve timing closure.
      mask init:
      | pipeline_init(gcb,'latency',latency);
      settings: AttributesFormatString=Latency = %<latency>
      mask Display:
      | port_label('input', 1, 'd');
      | port_label('output', 1, 'q');
      | disp(['Z^-', num2str(latency)]);
  pipeline3 : Subsystem  AncestorBlock=casper_library_delays/pipeline  mask(pipeline){latency=2}
      mask help:
      | An explicitly laid-out delay line to avoid mapping to SRL16s
      | for use in pipelining to help achieve timing closure.
      mask init:
      | pipeline_init(gcb,'latency',latency);
      settings: AttributesFormatString=Latency = %<latency>
      mask Display:
      | port_label('input', 1, 'd');
      | port_label('output', 1, 'q');
      | disp(['Z^-', num2str(latency)]);
  pipeline4 : Subsystem  AncestorBlock=casper_library_delays/pipeline  mask(pipeline){latency=2}
      mask help:
      | An explicitly laid-out delay line to avoid mapping to SRL16s
      | for use in pipelining to help achieve timing closure.
      mask init:
      | pipeline_init(gcb,'latency',latency);
      settings: AttributesFormatString=Latency = %<latency>
      mask Display:
      | port_label('input', 1, 'd');
      | port_label('output', 1, 'q');
      | disp(['Z^-', num2str(latency)]);
  pipeline5 : Subsystem  AncestorBlock=casper_library_delays/pipeline  mask(pipeline){latency=2}
      mask help:
      | An explicitly laid-out delay line to avoid mapping to SRL16s
      | for use in pipelining to help achieve timing closure.
      mask init:
      | pipeline_init(gcb,'latency',latency);
      settings: AttributesFormatString=Latency = %<latency>
      mask Display:
      | port_label('input', 1, 'd');
      | port_label('output', 1, 'q');
      | disp(['Z^-', num2str(latency)]);
  pipeline6 : Subsystem  AncestorBlock=casper_library_delays/pipeline  mask(pipeline){latency=2}
      mask help:
      | An explicitly laid-out delay line to avoid mapping to SRL16s
      | for use in pipelining to help achieve timing closure.
      mask init:
      | pipeline_init(gcb,'latency',latency);
      settings: AttributesFormatString=Latency = %<latency>
      mask Display:
      | port_label('input', 1, 'd');
      | port_label('output', 1, 'q');
      | disp(['Z^-', num2str(latency)]);
  pipeline7 : Subsystem  AncestorBlock=casper_library_delays/pipeline  mask(pipeline){latency=2}
      mask help:
      | An explicitly laid-out delay line to avoid mapping to SRL16s
      | for use in pipelining to help achieve timing closure.
      mask init:
      | pipeline_init(gcb,'latency',latency);
      settings: AttributesFormatString=Latency = %<latency>
      mask Display:
      | port_label('input', 1, 'd');
      | port_label('output', 1, 'q');
      | disp(['Z^-', num2str(latency)]);
  pipeline8 : Subsystem  AncestorBlock=casper_library_delays/pipeline  mask(pipeline){latency=4}
      mask help:
      | An explicitly laid-out delay line to avoid mapping to SRL16s
      | for use in pipelining to help achieve timing closure.
      mask init:
      | pipeline_init(gcb,'latency',latency);
      settings: AttributesFormatString=Latency = %<latency>
      mask Display:
      | port_label('input', 1, 'd');
      | port_label('output', 1, 'q');
      | disp(['Z^-', num2str(latency)]);
  pipeline9 : Subsystem  AncestorBlock=casper_library_delays/pipeline  mask(pipeline){latency=2}
      mask help:
      | An explicitly laid-out delay line to avoid mapping to SRL16s
      | for use in pipelining to help achieve timing closure.
      mask init:
      | pipeline_init(gcb,'latency',latency);
      settings: AttributesFormatString=Latency = %<latency>
      mask Display:
      | port_label('input', 1, 'd');
      | port_label('output', 1, 'q');
      | disp(['Z^-', num2str(latency)]);
  pkt_reord_devel : Subsystem  mask{ant_bits=n_bits_ants, xeng_bits=n_bits_xengs, chan_bits=n_bits_channels, x_int_bits=x_acc_bits, window_bits=5, min_sync_bits=8+(n_bits_channels-n_bits_xengs)+3, n_bits_flag=15, n_bits_timestamp=timestamp_bits, n_bits_data=32, n_bits_input_words=1, n_bits_output_words=0}
      mask prompts: ant_bits "Maximum Number of Antennas (2^?):"; xeng_bits "Number of Xengines in the system (2^?)"; chan_bits "Number of frequency channels in the system (2^?)"; x_int_bits "X Engine Integration Length (2^?):"; window_bits "Number of Windows to Buffer (2^?):"; min_sync_bits "Minimum sync period (2^n)"; n_bits_flag "Flag bit width"; n_bits_timestamp "Timestamp bit width"; n_bits_data "Input data word width"; n_bits_input_words "Input data words (2^?)"; n_bits_output_words "Output data words (2^?)"
      mask init:
      | sync_bits=max([min_sync_bits, (chan_bits-xeng_bits)+x_int_bits+ant_bits-n_bits_output_words]);
      | %sync_bits=chan_bits+x_int_bits+ant_bits-xeng_bits;
      | buf_bits=x_int_bits+ant_bits+window_bits-n_bits_input_words;
      | fmtstr = sprintf('Sync period: 2^%d\nPayload Len: %i', sync_bits, 2^(x_int_bits - 2));
      | set_param(gcb, 'AttributesFormatString', fmtstr);
      settings: AttributesFormatString=|
      | Sync period: 2^21
      | Payload Len: 64
  pre_process : Subsystem  mask{share_bits=0, xeng_bits=n_bits_xengs, freq_bits=n_bits_channels, acc_bits=x_acc_bits, time_bits=3, ant_bits=n_bits_ants}
      mask prompts: share_bits "Number of X-engines on this link (2^N)?"; xeng_bits "Number of X-engines in system (2^N)?"; freq_bits "Number of frequency channels in system (2^N)?"; acc_bits "xengine accumulation length (2^?)"; time_bits "samples per timestamp increment (2^?)"; ant_bits "max number of antennas in system (2^?)"
  speadify0 : Subsystem  mask(speadify){spead_msw=64, spead_lsw=48, heap_bits=n_bits_channels-n_bits_xengs+x_acc_bits, group_size_bits=n_bits_xengs, n_bits_chans=n_bits_channels-n_bits_xengs, n_bits_acc=x_acc_bits, bit_width_in=1, packet_bits=12, fabric_clock=225, tx_clock=156.25}
      mask prompts: spead_msw "SPEAD flavour (msw)"; spead_lsw "SPEAD flavour (lsw)"; heap_bits "heap size (2^? input words)"; group_size_bits "max SPEAD heap group size (2^?)"; n_bits_chans "channels processed (2^?)"; n_bits_acc "samples from channel (2^?)"; bit_width_in "word size in (2^? bytes)"; packet_bits "packet size out (2^? bytes)"; fabric_clock "fabric clock (MHz)"; tx_clock "transmission clock (MHz)"
      mask help:
      | Transforms input data stream to 10Ge ready SPEAD stream.
      | max SPEAD heap group size is the maximum number of SPEAD sources
      | that may be combined when assembling heaps. n_partitions and partition
      | input ports are then used at runtime to configure this.
  speadify1 : Subsystem  mask(speadify){spead_msw=64, spead_lsw=48, heap_bits=n_bits_channels-n_bits_xengs+x_acc_bits, group_size_bits=n_bits_xengs, n_bits_chans=n_bits_channels-n_bits_xengs, n_bits_acc=x_acc_bits, bit_width_in=1, packet_bits=12, fabric_clock=225, tx_clock=156.25}
      mask prompts: spead_msw "SPEAD flavour (msw)"; spead_lsw "SPEAD flavour (lsw)"; heap_bits "heap size (2^? input words)"; group_size_bits "max SPEAD heap group size (2^?)"; n_bits_chans "channels processed (2^?)"; n_bits_acc "samples from channel (2^?)"; bit_width_in "word size in (2^? bytes)"; packet_bits "packet size out (2^? bytes)"; fabric_clock "fabric clock (MHz)"; tx_clock "transmission clock (MHz)"
      mask help:
      | Transforms input data stream to 10Ge ready SPEAD stream.
      | max SPEAD heap group size is the maximum number of SPEAD sources
      | that may be combined when assembling heaps. n_partitions and partition
      | input ports are then used at runtime to configure this.
  tagger_and_flagger : Subsystem  mask{write_period=2^(n_bits_ants+8+n_bits_channels-n_bits_xengs), read_period=((2^n_bits_ants * ((2^n_bits_ants) + 1))/2) * 8 * (2^(n_bits_channels-n_bits_xengs-1)), n_bits_flags=ones(1,19)}
      mask prompts: write_period "input flag storage period"; read_period "output port flag storage period"; n_bits_flags "flag bit widths"
  take_off_zeros : xbsIndex_r4/Slice  nbits=32  boolean_output=off  mode=Two Bit Locations  bit1=0  base1=MSB of Input  bit0=n_bits_channels + 1 + x_acc_bits  base0=LSB of Input  dbl_ovrd=off  block_type=slice
  tl_reord_flags : Subsystem  mask(timed_latch){n_bits_time=48, n_bits_offset=8+(n_bits_channels-n_bits_xengs), n_bits_counters=8}
      mask prompts: n_bits_time "Total time resolution (bits)"; n_bits_offset "Offset from lsb for comparison"; n_bits_counters "Bits in status counters"
      mask help:
      | Latches load_value when armed and current_time matches requested time.
      | current_time should be in ADC samples.
      mask init:
      | set_param([gcb,'/status'], 'bitwidths', mat2str([1, repmat(n_bits_counters, 1, 2)]));
      mask Help:
      | When armed, will latch new value when current time matches the time
      | specified. The input time should be in samples and mask settings allow
      | a portion of this to be compared to cater for quantization. Arm and latch
      | counts allow the current state, pending and missed latch events to be
      | determined.
  vacc : Subsystem  Tag=casper:vacc  mask{ants_bits=n_bits_ants, freq_bits=n_bits_channels, xeng_bits=n_bits_xengs, acc_bits=x_acc_bits, tick_bits=0, which_qdr=qdr0, n_inputs=1, n_bits=32, n_bits_flags=ones(1,19)}
      mask prompts: ants_bits "Number of antennas (2^n)"; freq_bits "Number of frequency channels (2^n)"; xeng_bits "Number of X engines (2^n)"; acc_bits "Pre-accumulation in xengine (2^?)"; tick_bits "Timestamp samples per tick (2^?)"; which_qdr "QDR"; n_inputs "Simultaneous inputs (2^?)"; n_bits "Data width (bits)"; n_bits_flags "Flag bit widths"
      mask help: Hardcoded for X engines with a demux of 8!
      mask init:
      | vector_len = (2^ants_bits)*(2^ants_bits +1) /2 *8 * 2^(freq_bits-xeng_bits-n_inputs);
      | set_param([gcb, '/qv'], 'which_qdr', which_qdr);
      | fmtstr = sprintf('Vector Length: %d', vector_len);
      | set_param(gcb, 'AttributesFormatString', fmtstr);
      settings: AttributesFormatString=Vector Length: 147456
      mask TypeOptions which_qdr: qdr0 | qdr1 | qdr2 | qdr3
  vacc_tvg0 : Subsystem  AncestorBlock=casper_library/Accumulators/vacc_tvg  mask{len=(2^n_bits_ants*(2^n_bits_ants+1))/2*8*2^(n_bits_channels-n_bits_xengs-1), n_bits=32, n_inputs=2}
      mask prompts: len "Number of Vectors"; n_bits "Data bits"; n_inputs "Simultaneous inputs"
      mask init:
      | fmtstr = sprintf('Vector Length: %d', len);
      | set_param(gcb, 'AttributesFormatString', fmtstr);
      settings: AttributesFormatString=Vector Length: 147456
  vector_ctr : xbsIndex_r4/Counter  cnt_type=Free Running  cnt_to=Inf  operation=Up  start_count=0  cnt_by_val=1  arith_type=Unsigned  n_bits=13  bin_pt=0  load_pin=off  rst=on  en=on  explicit_period=on  period=1  dbl_ovrd=off  use_behavioral_HDL=off  implementation=Fabric  block_type=counter
  xeng : Subsystem  Tag=casper:xeng  AncestorBlock=casper_library_correlator/xeng  mask(xeng){n_ants=2^n_bits_ants, n_bits=8, acc_len=2^x_acc_bits, demux_factor=4, add_latency=3, mult_latency=4, bram_latency=7, use_ded_mult=1, use_bram_delay=1}
      mask prompts: n_ants "Number of antennas"; n_bits "Bit-width of samples in"; acc_len "Accumulation length"; add_latency "Adder latency"; mult_latency "Multiplier latency"; bram_latency "BRAM latency"; use_ded_mult "Implementation: Multiplier type (0=slices 1=embedded 2=bram)"; use_bram_delay "Implementation: Delay type (0=SLR, 1=BRAM)"
      mask help: CASPER X engine with added internal valid data masking functionality, descramble and integral demux. Based on Aaron Parsons' and Lynn Urry's original X engine design.
      mask init:
      | xeng_init(gcb, ...
      |     'n_ants', n_ants, ...
      |     'n_bits', n_bits, ...
      |     'acc_len', acc_len, ...
      |     'demux_factor', demux_factor, ...
      |     'add_latency', add_latency, ...
      |     'mult_latency', mult_latency, ...
      |     'bram_latency', bram_latency, ...
      |     'use_ded_mult', use_ded_mult, ...
      |     'use_bram_delay', use_bram_delay);
      settings: AttributesFormatString=n_ant=8, bits=8, mult_typ=1, bram_typ=1
      mask TypeOptions demux_factor: 1 | 2 | 4 | 8
  xeng_tvg : Subsystem  AncestorBlock=casper_library/Correlator/xeng_tvg  mask{n_bits=8, ant_bits=n_bits_ants, x_int_bits=x_acc_bits, sync_period=8+(n_bits_channels-n_bits_xengs)+4, mcnt_period=8+(n_bits_channels-n_bits_xengs), mcnt_step=(n_bits_channels+1-3)+8, n_bits_mcnt=timestamp_bits}
      mask prompts: n_bits "Data bits"; ant_bits "Number of Antennas (2^?):"; x_int_bits "X Integration Length (2^?):"; sync_period "Sync Pulse Period (2^?):"; mcnt_period "Mcnt period (2^?)"; mcnt_step "Mcnt step (2^?)"; n_bits_mcnt "Mcnt bit width (2^?)"
  zeros : Subsystem  AncestorBlock=casper_library_bus/bus_constant  mask(bus_constant){values=zeros(1,19), n_bits=ones(1,19), bin_pts=0, types=0}
      mask prompts: n_bits "bit widths"; bin_pts "binary points"; types "data type"
      mask help: Combine constants into a bus
      mask init:
      | bus_constant_init(gcb, ...
      |     'values', values, ...
      |     'n_bits', n_bits, ...
      |     'bin_pts', bin_pts, ...
      |     'types', types);
  tag scope: accumulating0=global, bf0s_d0=global, bf0s_en0=global, bf0s_eof0=global, bf0s_of0=global, bf0s_pkt_ready0=global, bf1s_d0=global, bf1s_en0=global, bf1s_eof0=global, bf1s_of0=global, bf1s_pkt_ready0=global, bfout_d0=global, bfout_den0=global, bfout_sync0=global, bfout_time0=global, bfout_valbw0=global, bfout_valfilt0=global, bfout_valquant0=global, flags_error0=global, flags_warning0=global, id0=global, pack_err0=global, pack_fetch0=global, pack_ready0=global, pack_txd0=global, pack_txeof0=global, pack_txvld0=global, pre_adc_err0=global, pre_data_0=global, pre_eof_0=global, pre_feng_chk_err0=global, pre_feng_id_0=global, pre_feng_qdr_err0=global, pre_feng_rx_err0=global, pre_fft_err0=global, pre_freq_0=global, pre_ndiode_en0=global, pre_rx_dest_err0=global, pre_spead_err0=global, pre_timestamp_0=global, pre_valid_0=global, reord_data0=global, reord_flag0=global, reord_freq0=global, reord_pktdisc0=global, reord_recv0=global, reord_recverr0=global, reord_sync0=global, reord_time0=global, reord_timeouterr0=global, reord_valid0=global, tf_data0=global, tf_flag0=global, tf_sync0=global, tf_valid0=global, vacc_data0=global, vacc_err0=global, vacc_err_flags0=global, vacc_flag0=global, vacc_ld_stat0=global, vacc_newacc0=global, vacc_pktrdy0=global, vacc_rbdone0=global, vacc_time0=global, vacc_valid0=global, vaccin_arm0=global, vaccin_data0=global, vaccin_flags0=global, vaccin_rst0=global, vaccin_sync0=global, vaccin_time0=global, vaccin_valid0=global, xeng_acc64_0=global, xeng_dv_0=global, xeng_mcnt27_0=global, xeng_sync_0=global
  wires:
  [pre_valid_0] -> Delay1/2, Delay5/2, Delay4/2, Delay3/2, Delay2/2, Delay6/1
  [pre_eof_0] -> Delay7/1
  [id0] -> pkt_reord_devel/8(board_id)
  pkt_reord_devel/1(sync_out) -> Delay20/1(d)
  pkt_reord_devel/2(data_out) -> Delay15/1(d)
  pkt_reord_devel/3(valid_out) -> Logical1/2, Delay16/1(d)
  pkt_reord_devel/4(time_out) -> Delay18/1(d)
  pkt_reord_devel/5(freq_out) -> Delay23/1(d)
  pkt_reord_devel/6(flags_out) -> Delay19/1(d)
  pkt_reord_devel/8(packet_discarded) -> Delay22/1(d)
  Delay20/1(q) -> [reord_sync0]
  Delay15/1(q) -> [reord_data0]
  Delay16/1(q) -> [reord_valid0]
  Delay18/1(q) -> [reord_time0]
  Delay23/1(q) -> [reord_freq0]
  Delay19/1(q) -> [reord_flag0]
  Delay22/1(q) -> [reord_pktdisc0]
  Delay89/1(q) -> [reord_timeouterr0]
  pkt_reord_devel/9(mcnt_timeout) -> Delay89/1(d)
  Delay1/1 -> pkt_reord_devel/1(din)
  Delay5/1 -> pkt_reord_devel/7(flags_in)
  Delay3/1 -> pkt_reord_devel/5(ant)
  Delay4/1 -> pkt_reord_devel/6(freq)
  Delay2/1 -> pkt_reord_devel/4(time)
  [pre_timestamp_0] -> Delay2/1
  [pre_data_0] -> Delay1/1
  [pre_feng_id_0] -> Delay3/1
  [pre_freq_0] -> Delay4/1
  Delay6/1 -> pkt_reord_devel/2(valid_in)
  Delay7/1 -> pkt_reord_devel/3(eof)
  pkt_reord_devel/7(recvd) -> Inverter/1, Delay21/1(d)
  Inverter/1 -> Logical1/1
  Logical1/1 -> Delay8/1(d)
  Delay21/1(q) -> [reord_recv0]
  Delay8/1(q) -> [reord_recverr0]
  [xeng_tvg_sel] -> xeng_tvg/1(tvg_sel)
  [reord_sync0] -> xeng_tvg/2(sync)
  [reord_data0] -> xeng_tvg/3(data_in)
  [reord_valid0] -> xeng_tvg/4(valid_in)
  [reord_time0] -> xeng_tvg/5(mcnti)
  Concat2/1 -> xeng_tvg/6(misci)
  Delay84/1(q) -> [xin_sync0]
  Delay78/1(q) -> [xin_data0]
  Delay79/1(q) -> [xin_valid0]
  Delay83/1(q) -> [xin_time0]
  Delay111/1(q) -> [xin_flag0]
  tagger_and_flagger/2(output_data_out) -> Delay10/1(d)
  [xin_sync0] -> xeng/1(sync_in), tagger_and_flagger/1(input_sync)
  [xin_data0] -> xeng/2(ant)
  [xin_valid0] -> xeng/3(window_valid), tagger_and_flagger/2(input_en)
  [xin_time0] -> xeng/4(mcnt_in), tagger_and_flagger/3(tag_in)
  tagger_and_flagger/1(output_sync_out) -> Delay9/1(d)
  tagger_and_flagger/3(output_dvalid) -> Delay11/1(d)
  Concat13/1 -> Delay12/1(d)
  [xin_flag0] -> tagger_and_flagger/4(flag_in), bus_relational/2(b)
  zeros/1(dout) -> bus_relational/1(a)
  bus_relational/1(a!=b) -> tagger_and_flagger/5(flag_sample)
  tagger_and_flagger/4(tag_out) -> Concat13/1
  tagger_and_flagger/5(flag_out) -> Concat13/2
  [vacc_tvg_sel] -> vacc_tvg0/1(tvg_sel)
  pipeline/1(q) -> [vacc_data0]
  pipeline1/1(q) -> [vacc_valid0]
  pipeline2/1(q) -> [vacc_rbdone0]
  pipeline3/1(q) -> [vacc_time0]
  [vacc_ld_immediate] -> vacc/4(immediate)
  [vacc_rst] -> vacc/1(rst), [vaccin_rst0]
  [vacc_ld_time] -> Slice1/1
  [vacc_ld_arm] -> vacc/2(arm), [vaccin_arm0]
  [acc_len] -> vacc/5(acc_len)
  vacc_tvg0/3(valid_out) -> [vaccin_valid0], pipeline7/1(d)
  vacc_tvg0/1(sync_out) -> pipeline5/1(d), [vaccin_sync0]
  vacc_tvg0/4(misco) -> bus_expand2/1(bus_in)
  pipeline4/1(q) -> [vacc_flag0]
  vacc/11(error_out) -> [vacc_err0]
  [tf_valid0] -> vacc_tvg0/4(valid_in)
  [tf_data0] -> vacc_tvg0/3(data_in)
  [tf_flag0] -> vacc_tvg0/5(misci)
  [tf_sync0] -> vacc_tvg0/2(sync_in)
  [pack_fetch0] -> vacc/11(re)
  vacc/10(fifo_afull) -> Terminator5/1
  pack_out/3(eof) -> Delay69/1(d)
  [vacc_data0] -> pack_out/1(data_in)
  [vacc_valid0] -> pack_out/2(valid_in)
  [vacc_rbdone0] -> pack_out/4(rb_done)
  pack_out/1(data_out) -> Delay74/1(d)
  pack_out/4(err) -> Delay76/1(d)
  Delay76/1(q) -> [pack_err0]
  Delay69/1(q) -> [pack_txeof0], Register/2
  Delay74/1(q) -> [pack_txd0]
  [gbe_txen] -> Register/1
  Register/1 -> Logical/1
  pack_out/2(valid_out) -> Delay77/1(d)
  Logical/1 -> [pack_txvld0]
  Delay77/1(q) -> Logical/2
  pack_out/6(pkt_ready) -> [pack_ready0]
  [vacc_pktrdy0] -> pack_out/3(pkt_rdy)
  [id0] -> pack_out/7(xeng_id)
  [go0] -> pack_out/8(go)
  pack_out/5(fetch) -> [pack_fetch0]
  bus_expand2/1(msb_out2) -> pipeline10/1(d), [vaccin_time0]
  Delay9/1(q) -> [tf_sync0]
  Delay10/1(q) -> [tf_data0]
  Delay11/1(q) -> [accumulating0], [tf_valid0]
  Delay12/1(q) -> [tf_flag0]
  [vaccin_valid0] -> Logical3/2, vector_ctr/2
  Logical2/1 -> vector_ctr/1
  vector_ctr/1 -> Relational1/1, Relational/1  "vec_ctr"
  Slice/1 -> Relational/2
  Constant3/1 -> Concat4/1
  Constant4/1 -> Concat4/2
  Concat4/1 -> Mux1/3
  Constant1/1 -> Mux1/2
  Mux1/1 -> Terminator1/1  "tvgdata"
  Relational1/1 -> Logical2/2  "vec_done"
  Constant6/1 -> Relational1/2
  Logical3/1 -> Mux1/1  "prodsel"
  Constant7/1 -> Register1/1
  [vaccin_sync0] -> Register1/2, Logical2/1
  Relational/1 -> Logical3/3  "prodsel"
  Register1/1 -> Logical3/1
  [vaccin_newtvg] -> Slice/1
  vacc_tvg0/2(data_out) -> pipeline6/1(d), [vaccin_data0]
  flags/1(flagso) -> pack_out/6(flags)
  [vacc_flag0] -> Concat/1
  [vacc_err0] -> Concat/2
  Concat/1 -> flags/1(flagsi)
  pipeline5/1(q) -> vacc/6(sync_in)
  pipeline6/1(q) -> vacc/7(data_in)
  pipeline7/1(q) -> vacc/8(we)
  pipeline9/1(q) -> vacc/10(flags_in)
  pipeline10/1(q) -> vacc/9(timestamp_in)
  [spead_data0] -> Delay13/1(d)
  [spead_valid0] -> Delay14/1(d)
  [spead_eof0] -> Delay17/1(d)
  [spead_error0] -> Delay24/1(d)
  [spead_hdr1_0] -> Delay25/1(d)
  [spead_hdr2_0] -> Delay26/1(d)
  [id0] -> Delay29/1(d)
  [spead_error0] -> Concat2/4
  [reord_pktdisc0] -> Concat2/3
  [reord_recverr0] -> Concat2/2
  [reord_flag0] -> Concat2/5
  [reord_timeouterr0] -> Concat2/1
  vacc/12(error_flags) -> [vacc_err_flags0]
  vacc/1(new_acc) -> [vacc_newacc0]
  vacc/2(data_out) -> pipeline/1(d)
  vacc/3(oob_out) -> Terminator4/1
  vacc/4(valid_out) -> pipeline1/1(d)
  vacc/5(pkt_rdy) -> [vacc_pktrdy0]
  vacc/6(rb_done) -> pipeline2/1(d)
  vacc/7(timestamp_out) -> pipeline3/1(d)
  vacc/8(flags_out) -> pipeline4/1(d)
  vacc/9(start_status) -> [vacc_ld_stat0]
  [gap_size0] -> pack_out/9(gap_size)
  xeng_tvg/1(sync_out) -> Concat5/1
  Constant9/1 -> Concat3/2
  Constant8/1 -> tl_reord_flags/1(rst)
  xeng_tvg/3(valid_out) -> tl_reord_flags/4(en)
  Concat5/1 -> tl_reord_flags/5(misci)
  xeng_tvg/2(data_out) -> Concat5/2
  xeng_tvg/5(misco) -> Concat5/3
  Constant2/1 -> tl_reord_flags/3(load_value)
  tl_reord_flags/3(dvalid) -> flag_mux/3(en)
  [flags0] -> flag_mux/6(tvg_flag)
  tl_reord_flags/1(value) -> Terminator/1
  tl_reord_flags/2(enable) -> flag_mux/2(ld_val)
  tl_reord_flags/5(misco) -> bus_expand20/1(bus_in)
  bus_expand20/2(lsb_out1) -> flag_mux/5(flag)
  Concat7/1 -> flag_mux/4(misci)
  bus_expand20/1(msb_out2) -> Concat7/2
  tl_reord_flags/4(time) -> take_off_zeros/1
  [tvg_flags_sel0] -> flag_mux/1(tvg_en)
  Concat3/1 -> tl_reord_flags/2(current_time)
  xeng_tvg/4(mcnto) -> Concat3/1
  flag_mux/2(misco) -> bus_expand1/1(bus_in)
  bus_expand1/1(msb_out3) -> Delay83/1(d)
  bus_expand1/2(out2) -> Delay84/1(d)
  bus_expand1/3(lsb_out1) -> Delay78/1(d)
  flag_mux/3(flags_out) -> Delay111/1(d)
  flag_mux/1(dvalid) -> Delay79/1(d)
  Delay13/1(q) -> pre_process/1(data_in)
  Delay14/1(q) -> pre_process/2(valid_in)
  Delay17/1(q) -> pre_process/3(eof_in)
  Delay26/1(q) -> pre_process/6(spead_fengid)
  Delay24/1(q) -> pre_process/4(spead_err)
  Delay25/1(q) -> pre_process/5(spead_time48)
  Delay28/1(q) -> pre_process/8(heap_offset)
  Delay27/1(q) -> pre_process/7(spead_flags)
  Constant10/1 -> Concat6/2
  Slice11/1 -> Concat6/1
  Concat6/1 -> [id0]
  [board_id] -> Slice11/1
  bus_expand2/2(lsb_out1) -> [vaccin_flags0], pipeline9/1(d)
  Delay29/1(q) -> pre_process/9(xeng_id)
  xeng/1(sync_out) -> [xeng_sync_0], tagger_and_flagger/6(output_sync_in)
  xeng/4(mcnt_out) -> [xeng_mcnt27_0]
  xeng/3(acc) -> tagger_and_flagger/7(output_data_in), [xeng_acc64_0]
  xeng/2(valid) -> [xeng_dv_0], tagger_and_flagger/8(output_en)
  Constant11/1 -> bf/4(badi)
  Constant12/1 -> bf/6(misci)
  Slice2/1 -> speadify0/3(di)
  bf/5(misco) -> pipeline17/1(d)
  [reord_sync0] -> Delay35/1(d)
  [reord_valid0] -> Delay37/1(d)
  bf/3(deno) -> pipeline13/1(d)
  bf/2(do) -> pipeline11/1(d)
  Register2/1 -> [bf0s_d0]
  Delay68/1 -> [bf0s_eof0], Register5/2
  Delay71/1 -> [bf0s_pkt_ready0]
  [bf0_tx_pkt0] -> speadify0/6(start)
  Slice15/1 -> speadify0/4(eni)
  speadify0/1(do) -> Register2/1
  speadify0/2(eno) -> Delay93/1, Register2/2
  speadify0/3(eofo) -> Delay68/1
  speadify0/4(pkt_ready) -> Delay71/1
  speadify0/5(of) -> Delay30/1
  [bf0_rst] -> speadify0/1(rst)
  Delay30/1 -> [bf0s_of0]
  [id0] -> speadify0/7(id)
  Register3/1 -> [bf1s_d0]
  Delay32/1 -> [bf1s_eof0], Register4/2
  Delay33/1 -> [bf1s_pkt_ready0]
  bf/4(timeo) -> pipeline12/1(d)
  speadify1/1(do) -> Register3/1
  speadify1/2(eno) -> Delay34/1, Register3/2
  speadify1/3(eofo) -> Delay32/1
  speadify1/4(pkt_ready) -> Delay33/1
  speadify1/5(of) -> Delay31/1
  [bf1_rst] -> speadify1/1(rst)
  Delay31/1 -> [bf1s_of0]
  bf/1(synco) -> pipeline8/1(d)
  Slice12/1 -> speadify1/3(di)
  Delay38/1(q) -> bf/5(timei)
  [reord_time0] -> Delay38/1(d)
  [id0] -> Delay39/1(d)
  Delay39/1(q) -> bf/7(beng_id)
  Delay37/1(q) -> bf/3(deni)
  Delay35/1(q) -> bf/1(synci)
  bf/6(value_out_bw) -> pipeline14/1(d)
  bf/7(value_out_quant) -> pipeline16/1(d)
  bf/8(value_out_filt) -> pipeline15/1(d)
  [bfout_sync0] -> speadify1/2(synci), speadify0/2(synci)
  [bfout_d0] -> Slice12/1, Slice2/1
  [bfout_den0] -> Slice16/1, Slice15/1
  [bfout_time0] -> speadify1/5(timei), speadify0/5(timei)
  pipeline8/1(q) -> [bfout_sync0]
  pipeline11/1(q) -> [bfout_d0]
  pipeline13/1(q) -> [bfout_den0]
  pipeline17/1(q) -> Terminator2/1
  pipeline14/1(q) -> [bfout_valbw0]
  pipeline15/1(q) -> [bfout_valfilt0]
  pipeline16/1(q) -> [bfout_valquant0]
  [bf1_txen] -> Register4/1
  Register4/1 -> Logical4/1
  Logical4/1 -> [bf1s_en0]
  [bf0_txen] -> Register5/1
  Register5/1 -> Logical5/1
  Logical5/1 -> [bf0s_en0]
  Delay34/1 -> Logical4/2
  Delay36/1(q) -> [pre_data_0]
  Delay40/1(q) -> [pre_valid_0]
  Delay41/1(q) -> [pre_eof_0]
  Delay42/1(q) -> [pre_timestamp_0]
  Delay43/1(q) -> [pre_feng_id_0]
  Delay44/1(q) -> [pre_freq_0]
  Delay46/1(q) -> [pre_spead_err0]
  Delay48/1(q) -> Delay5/1
  Delay47/1(q) -> [pre_rx_dest_err0]
  [reord_data0] -> Mux/2
  Concat11/1 -> Mux/3
  [bf_tvgsel] -> Delay52/1(d)
  Delay52/1(q) -> Mux/1
  Mux/1 -> bf/2(di)
  Constant13/1 -> Concat10/2
  pipeline12/1(q) -> Concat10/1
  Concat10/1 -> [bfout_time0]
  take_off_zeros/1 -> Concat7/1
  Constant14/1 -> Concat11/3
  [reord_freq0] -> Concat11/2
  Constant15/1 -> Concat11/1
  Slice1/1 -> vacc/3(start_time)
  Constant5/1 -> Concat1/2
  Concat1/1 -> pack_out/5(timestamp)
  [vacc_time0] -> Concat1/1
  flags/2(error) -> [flags_error0]
  flags/3(warning) -> [flags_warning0]
  Delay49/1(q) -> bus_expand3/1(bus_in)
  bus_expand3/1(msb_out6) -> [pre_feng_chk_err0]
  bus_expand3/2(out5) -> [pre_feng_qdr_err0]
  bus_expand3/3(out4) -> [pre_fft_err0]
  bus_expand3/4(out3) -> [pre_feng_rx_err0]
  bus_expand3/5(out2) -> [pre_adc_err0]
  bus_expand3/6(lsb_out1) -> [pre_ndiode_en0]
  Constant16/1 -> Delay27/1(d)
  [spead_heap_offset0] -> Delay28/1(d)
  Delay50/1(q) -> pre_process/10(freq_offset)
  [spead_hdr3_0] -> Delay50/1(d)
  pre_process/1(data_out) -> Delay36/1(d)
  pre_process/2(valid) -> Delay40/1(d)
  pre_process/3(eof_out) -> Delay41/1(d)
  pre_process/4(timestamp) -> Delay42/1(d)
  pre_process/5(feng_id) -> Delay43/1(d)
  pre_process/6(freq_out) -> Delay44/1(d)
  pre_process/7(spead_err_out) -> Delay46/1(d)
  pre_process/8(ip_dest_err) -> Delay47/1(d)
  pre_process/9(flags_out) -> Delay48/1(d)
  pre_process/10(err_bundle) -> Delay49/1(d)
  Slice16/1 -> speadify1/4(eni)
  [bf1_tx_pkt0] -> speadify1/6(start)
  [id0] -> speadify1/7(id)
  Delay93/1 -> Logical5/2
